simulink model "USV_SAR_GNSS"  (R2026b)
settings: Solver=VariableStepAuto  StopTime=600
undefined symbols (not defined in the file): arrival_dwell_time, arrival_radius, arrival_speed, assistance_duration, battery_capacity_J, battery_initial_soc, battery_return_soc, current_bias_x, current_bias_y, current_change_time, current_estimation_tau, current_x, current_y, drag_r, drag_u, F_max, gnss_bias_x, gnss_bias_y, gnss_loss_enabled, gnss_loss_end, gnss_loss_start, gnss_position_sigma, gnss_sample_time, home_x, home_y, inertia_z, initial_heading, initial_x, initial_y, integral_activation_radius, K_aw, K_distance, Kd_heading, Ki_position, Ki_u, Kp_heading, Kp_u, M_max, mass_usv, mob_contact_loss_enabled, mob_contact_loss_end, mob_contact_loss_start, mob_drift_change_enabled, mob_drift_change_time, mob_drift_factor_after, mob_position_sigma, mob_sensor_sample_time, mob_track_alpha, mob_track_beta, mob_track_max_age, mob_track_sample_time, nav_alpha, nav_beta, nav_max_prediction_time, nav_sample_time, num_waypoints, P_aux, P_thrust_max, P_turn_max, position_integral_limit ... (+6)
libraries: simulink x7
(part 2 of 2)

== stateflow chart USV_SAR_GNSS/Mission_Management/Route_Manager ==
  state Following_Route
    entry:
    waypoint_index = 1;
    x_target = waypoints(waypoint_index, 1);
    y_target = waypoints(waypoint_index, 2);
    final_waypoint = (waypoint_index == num_waypoints);
    during:
    if nav_valid && waypoint_index < num_waypoints && ...
    (x_target-x)^2 + (y_target-y)^2 <= arrival_radius^2
    waypoint_index = waypoint_index + 1;
    end
    x_target = waypoints(waypoint_index, 1);
    y_target = waypoints(waypoint_index, 2);
    final_waypoint = (waypoint_index == num_waypoints);
  (default) -> Following_Route
  data: x input; y input; x_target output; y_target output; final_waypoint output; arrival_radius parameter; waypoints parameter; num_waypoints parameter size=1; waypoint_index output size=1; nav_valid input

== stateflow chart USV_SAR_GNSS/Mission_Management/SAR_Mission_Manager ==
  state Searching
    entry:
    target_found = false;
    mission_status = 0;
    assistance_completed = false;
    return_home=false;
    mission_completed=false;
    return_reason=0;
  state Approaching
    entry:
    target_found = true;
    mission_status = 1;
  state Search_Completed
    entry:
    target_found = false;
    mission_status = 3;
  state On_Scene
    entry:
    target_found = true;
    mission_status = 2;
    during:
    if contact_valid && ~(abort_mission || battery_low) && ...
    after(assistance_duration,sec)
    assistance_completed = true;
    end
  state Home_Reached
    entry:
    return_home=true;
    mission_status=5;
    mission_completed=true;
  state Returning_Home
    entry:
    return_home=true;
    mission_status=4;
    if battery_low
    return_reason=4;
    elseif abort_mission
    return_reason=3;
    elseif assistance_completed
    return_reason=1;
    else
    return_reason=2;
    end
  (default) -> Searching
  Searching -> Returning_Home [order 2] : [(abort_mission || battery_low)]
  Searching -> Search_Completed [order 3] : [~(abort_mission || battery_low) && route_final==1 && arrived==1 && ~target_detected]
  Searching -> Approaching [order 1] : [~(abort_mission || battery_low)&& target_detected]
  Search_Completed -> Approaching [order 1] : [~(abort_mission || battery_low) && target_detected]
  Approaching -> Returning_Home [order 2] : [(abort_mission || battery_low)]
  On_Scene -> Approaching [order 1] : [~(abort_mission || battery_low) && (~contact_valid || arrived==0)]
  Approaching -> On_Scene [order 1] : [~(abort_mission || battery_low) && contact_valid && arrived==1]
  Search_Completed -> Returning_Home [order 2] : [(abort_mission || battery_low) || ~target_detected]
  Returning_Home -> Home_Reached : [arrived==1 && (x-home_x)^2+(y-home_y)^2 <= arrival_radius^2]
  On_Scene -> Returning_Home [order 3] : [(abort_mission || battery_low)]
  On_Scene -> Returning_Home [order 2] : [~(abort_mission || battery_low) && assistance_completed && arrived==1]
  data: target_detected input boolean; target_found output boolean; arrived input; mission_status output; route_final input; assistance_duration parameter; assistance_completed output; return_home output; x input; y input; home_x parameter; home_y parameter; arrival_radius parameter; mission_completed output; abort_mission input; return_reason output; battery_low input; contact_valid input

== stateflow chart USV_SAR_GNSS/Mission_Management/Arrival_Manager ==
  state Navigating
    entry:
    arrived = 0;
  state Settling
    entry:
    arrived = 0;
  state Confirming
    entry:
    arrived = 0;
  state Arrived
    entry:
    arrived = 1;
  (default) -> Navigating
  Confirming -> Navigating [order 3] : [~nav_valid || final_waypoint == 0 || target_changed]
  Arrived -> Navigating [order 2] : [~nav_valid || target_changed]
  Settling -> Navigating [order 2] : [~nav_valid || final_waypoint == 0 || target_changed]
  Navigating -> Settling : [nav_valid && ~target_changed && final_waypoint == 1 && distance_to_target <= arrival_radius]
  Arrived -> Settling [order 1] : [nav_valid && (distance_to_target > 2*arrival_radius || relative_speed > 2*arrival_speed)]
  Confirming -> Settling [order 1] : [nav_valid && (distance_to_target > arrival_radius || relative_speed > arrival_speed)]
  Settling -> Confirming [order 1] : [nav_valid && distance_to_target <= arrival_radius && relative_speed <= arrival_speed]
  Confirming -> Arrived [order 2] : [nav_valid && after(arrival_dwell_time,sec) && distance_to_target <= arrival_radius && relative_speed <= arrival_speed]
  data: distance_to_target input; relative_speed input; arrived output; final_waypoint input; arrival_speed parameter; arrival_radius parameter; arrival_dwell_time parameter; target_changed input; nav_valid input
